simulink model "task1_simulation"  (R2025b)
settings: Solver=FixedStepAuto  StartTime=0.0  StopTime=40  RelTol=1e-3
undefined symbols (not defined in the file): d, DiscIntNeverNeededParam, is_real_robot, k_theta, k_x, k_y, q_goal_task1, q_goal_task2, q_init, r, Ts, X, Y
libraries: robotlib x6, sharedtransform x1
settings Model: Creator=dallaliber  LastModifiedBy=ilia
settings OptimizationCC: DefaultParameterBehavior=Inlined  EnhancedBackFolding=on  PassReuseOutputArgsAs=Individual arguments  ZeroExternalMemoryAtStartup=off  ZeroInternalMemoryAtStartup=off  MaxStackSize=64  OptimizeBlockOrder=speed  DifferentSizesBufferReuse=on  OptimizationCustomize=off  EfficientTunableParamExpr=on
settings DebuggingCC: ParameterTunabilityLossMsg=error
settings HardwareCC: ProdBitPerPointer=32.0  ProdBitPerSizeT=32.0  ProdBitPerPtrDiffT=32.0  ProdLargestAtomicFloat=None  ProdIntDivRoundTo=Undefined  ProdEndianess=Unspecified  ProdWordSize=32.0  ProdHWDeviceType=Generic->Unspecified (assume 32-bit Generic)
settings SFSimCC: MATLABDynamicMemAlloc=off
settings RTWCC: SystemTargetFile=ert.tlc  HardwareBoard=Robot Operating System (ROS)  TLCOptions="-aInlineSetEventsForThisBaseRateFcn=TLC_FALSE -aSuppressMultiTaskScheduler=TLC_FALSE  -aRateBasedStepFcn=0"  TemplateMakefile=ert_default_tmf  Toolchain=Catkin  TargetLang=C++  Description=Embedded Coder
settings CodeAppCC: ForceParamTrailComments=on  IgnoreCustomStorageClasses=off  OperatorAnnotations=on  SimulinkDataObjDesc=on  SFDataObjDesc=on  InsertBlockDesc=on
settings ERTTargetCC: DynamicArrayContainerType=coder::array

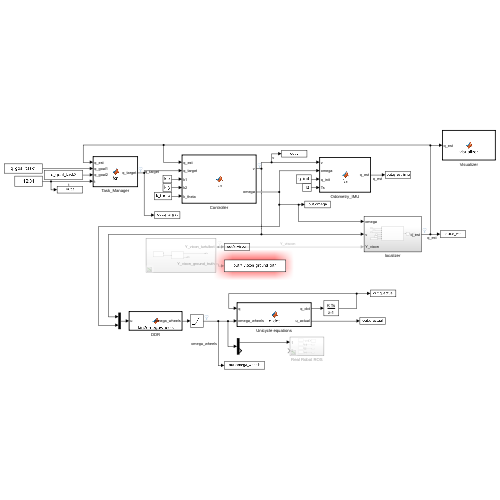
[thumbnail: Simulink's stored preview of the top-level diagram]
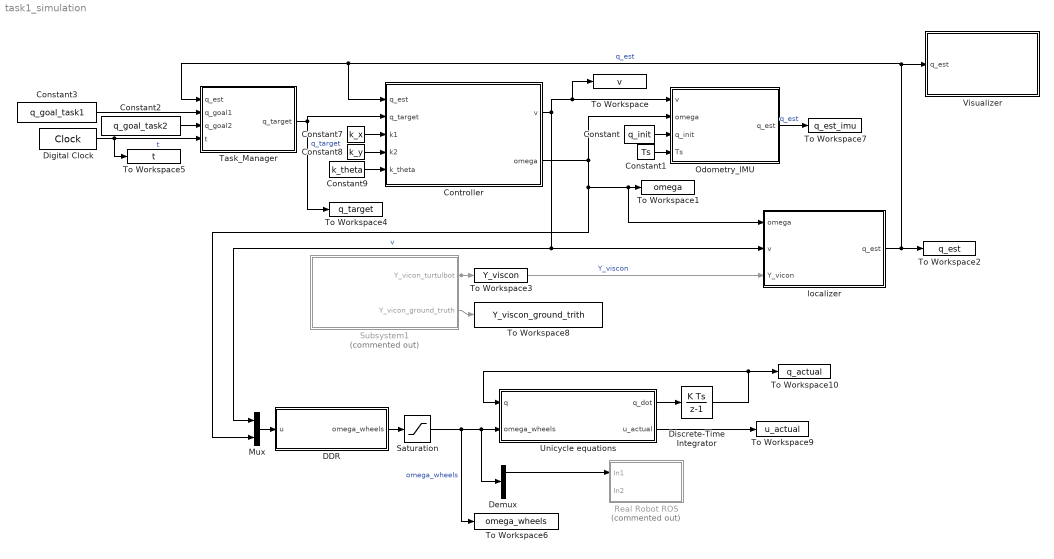
== system task1_simulation ==
  Constant : Constant  Value=q_init  SampleTime=Ts
  Constant1 : Constant  Value=Ts  SampleTime=Ts
  Constant2 : Constant  Value=q_goal_task2  SampleTime=Ts
  Constant3 : Constant  Value=q_goal_task1  SampleTime=Ts
  Constant7 : Constant  Value=k_x  SampleTime=Ts
  Constant8 : Constant  Value=k_y  SampleTime=Ts
  Constant9 : Constant  Value=k_theta  SampleTime=Ts
  Controller : MATLAB Function  TreatAsAtomicUnit=on
  DDR : MATLAB Function  TreatAsAtomicUnit=on
  Demux : Demux  Outputs=2
  Digital Clock : DigitalClock  SampleTime=Ts
  Discrete-Time Integrator : DiscreteIntegrator  InitialCondition=q_init  SampleTime=Ts  ICPrevOutput=DiscIntNeverNeededParam  ICPrevScaledInput=DiscIntNeverNeededParam
  Mux : Mux  Inputs=2
  Odometry_IMU : MATLAB Function  TreatAsAtomicUnit=on
  Real Robot ROS : Subsystem  Commented=on
  Saturation : Saturate  UpperLimit=10  LowerLimit=-10
  Subsystem1 : Subsystem  Commented=on
  Task_Manager : MATLAB Function  TreatAsAtomicUnit=on
  To Workspace : ToWorkspace  VariableName=v  SampleTime=Ts
  To Workspace1 : ToWorkspace  VariableName=omega  SampleTime=Ts
  To Workspace10 : ToWorkspace  VariableName=q_actual  SampleTime=Ts
  To Workspace2 : ToWorkspace  VariableName=q_est  SampleTime=Ts
  To Workspace3 : ToWorkspace  VariableName=Y_viscon  SampleTime=Ts
  To Workspace4 : ToWorkspace  VariableName=q_target  SampleTime=Ts
  To Workspace5 : ToWorkspace  VariableName=t  SampleTime=Ts
  To Workspace6 : ToWorkspace  VariableName=omega_wheels  SampleTime=Ts
  To Workspace7 : ToWorkspace  VariableName=q_est_imu  SampleTime=Ts
  To Workspace8 : ToWorkspace  VariableName=Y_viscon_ground_trith  SampleTime=Ts
  To Workspace9 : ToWorkspace  VariableName=u_actual  SampleTime=Ts
  Unicycle equations : MATLAB Function  TreatAsAtomicUnit=on
  Visualizer : MATLAB Function  TreatAsAtomicUnit=on
  localizer : Subsystem
  wires:
  Controller/1(v) -> Mux/1, localizer/2(v), Odometry_IMU/1(v), To Workspace/1  "v"
  Constant/1 -> Odometry_IMU/3(q_init)
  Constant1/1 -> Odometry_IMU/4(Ts)
  Constant2/1 -> Task_Manager/3(q_goal2)
  Constant3/1 -> Task_Manager/2(q_goal1)
  Odometry_IMU/1(q_est) -> To Workspace7/1  "q_est"
  Saturation/1 -> To Workspace6/1, Unicycle equations/2(omega_wheels), Demux/1  "omega_wheels"
  DDR/1(omega_wheels) -> Saturation/1
  Demux/1 -> Real Robot ROS/1(In1)
  Mux/1 -> DDR/1(u)
  Digital Clock/1 -> To Workspace5/1, Task_Manager/4(t)  "t"
  localizer/1(q_est) -> To Workspace2/1, Controller/1(q_est), Task_Manager/1(q_est), Visualizer/1(q_est)  "q_est"
  Subsystem1/1(Y_vicon_turtulbot) -> localizer/3(Y_vicon), To Workspace3/1  "Y_viscon"
  Task_Manager/1(q_target) -> To Workspace4/1, Controller/2(q_target)  "q_target"
  Constant7/1 -> Controller/3(k1)
  Constant8/1 -> Controller/4(k2)
  Subsystem1/2(Y_vicon_ground_truth) -> To Workspace8/1
  Constant9/1 -> Controller/5(k_theta)
  Controller/2(omega) -> localizer/1(omega), To Workspace1/1, Mux/2, Odometry_IMU/2(omega)
  Unicycle equations/1(q_dot) -> Discrete-Time Integrator/1
  Discrete-Time Integrator/1 -> To Workspace10/1, Unicycle equations/1(q)
  Unicycle equations/2(u_actual) -> To Workspace9/1

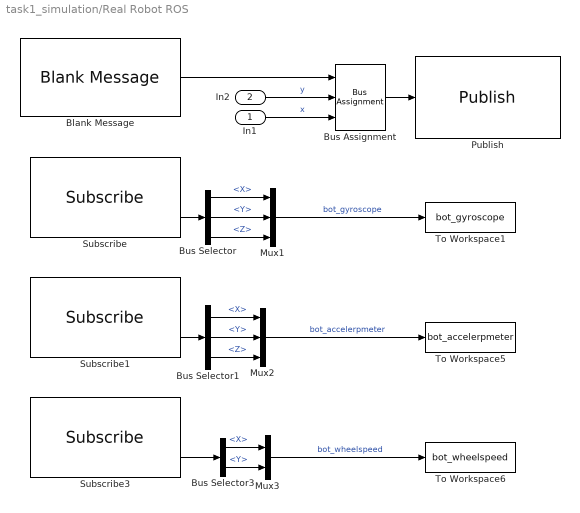
== system task1_simulation/Real Robot ROS ==
  In1 : Inport
  In2 : Inport  Port=2
  Blank Message : robotlib/Blank Message  messageClass=Message  entityType=geometry_msgs/Vector3  messageType=geometry_msgs/Vector3  SampleTime=0.04  legacyBusStruct=off
  Bus Assignment : BusAssignment  AssignedSignals=X,Y
  Bus Selector : BusSelector  OutputSignals=X,Y,Z
  Bus Selector1 : BusSelector  OutputSignals=X,Y,Z
  Bus Selector3 : BusSelector  OutputSignals=X,Y
  Mux1 : Mux  Inputs=3
  Mux2 : Mux  Inputs=3
  Mux3 : Mux  Inputs=2
  Publish : robotlib/Publish  topicSource=Select from ROS network  topic=/turtlebot_09/cmd_wheels  messageType=geometry_msgs/Vector3  legacyBusStruct=off  messageQueueLength=1
  Subscribe : robotlib/Subscribe  topicSource=Select from ROS network  topic=/turtlebot_09/gyroscope  messageType=geometry_msgs/Vector3  SampleTime=0.04  legacyBusStruct=off  messageQueueLength=1
  Subscribe1 : robotlib/Subscribe  topicSource=Select from ROS network  topic=/turtlebot_09/accelerometer  messageType=geometry_msgs/Vector3  SampleTime=0.04  legacyBusStruct=off  messageQueueLength=1
  Subscribe3 : robotlib/Subscribe  topicSource=Select from ROS network  topic=/turtlebot_09/wheelSpeeds  messageType=geometry_msgs/Vector3  SampleTime=0.04  legacyBusStruct=off  messageQueueLength=1
  To Workspace1 : ToWorkspace  VariableName=bot_gyroscope  SaveFormat=Timeseries  SampleTime=Ts
  To Workspace5 : ToWorkspace  VariableName=bot_accelerpmeter  SaveFormat=Timeseries  SampleTime=Ts
  To Workspace6 : ToWorkspace  VariableName=bot_wheelspeed  SaveFormat=Timeseries  SampleTime=Ts
  wires:
  Subscribe1/2 -> Bus Selector1/1
  Bus Selector1/1 -> Mux2/1  "<X>"
  Mux2/1 -> To Workspace5/1  "bot_accelerpmeter"
  Bus Assignment/1 -> Publish/1
  Subscribe/2 -> Bus Selector/1
  Bus Selector/2 -> Mux1/2  "<Y>"
  Bus Selector/1 -> Mux1/1  "<X>"
  Bus Selector3/1 -> Mux3/1  "<X>"
  Bus Selector3/2 -> Mux3/2  "<Y>"
  Bus Selector1/3 -> Mux2/3  "<Z>"
  Bus Selector1/2 -> Mux2/2  "<Y>"
  Mux3/1 -> To Workspace6/1  "bot_wheelspeed"
  Mux1/1 -> To Workspace1/1  "bot_gyroscope"
  Subscribe3/2 -> Bus Selector3/1
  Blank Message/1 -> Bus Assignment/1
  Bus Selector/3 -> Mux1/3  "<Z>"
  In1/1 -> Bus Assignment/3  "x"
  In2/1 -> Bus Assignment/2  "y"

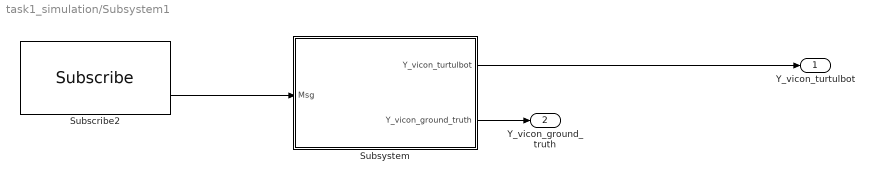
== system task1_simulation/Subsystem1 ==
  Subscribe2 : robotlib/Subscribe  topicSource=Select from ROS network  topic=/turtlebot_09/odom  messageType=nav_msgs/Odometry  SampleTime=Ts  legacyBusStruct=off  messageQueueLength=1
      settings: LibrarySourceBlock=roslib/ROS/Subscribe
  Subsystem : Subsystem
  Y_vicon_turtulbot : Outport
  Y_vicon_ground_truth : Outport  Port=2
  wires:
  Subscribe2/2 -> Subsystem/1(Msg)
  Subsystem/2(Y_vicon_ground_truth) -> Y_vicon_ground_truth/1
  Subsystem/1(Y_vicon_turtulbot) -> Y_vicon_turtulbot/1

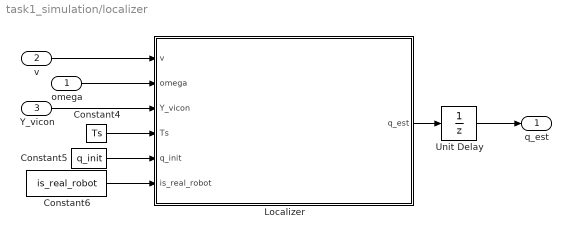
== system task1_simulation/localizer ==
  omega : Inport
  v : Inport  Port=2
  Y_vicon : Inport  Port=3
  Constant4 : Constant  Value=Ts
  Constant5 : Constant  Value=q_init
  Constant6 : Constant  Value=is_real_robot
  Localizer : MATLAB Function  TreatAsAtomicUnit=on
  Unit Delay : UnitDelay  InitialCondition=q_init  SampleTime=Ts  HasFrameUpgradeWarning=on
  q_est : Outport
  wires:
  Constant6/1 -> Localizer/6(is_real_robot)
  Y_vicon/1 -> Localizer/3(Y_vicon)
  Localizer/1(q_est) -> Unit Delay/1
  omega/1 -> Localizer/2(omega)
  Constant4/1 -> Localizer/4(Ts)
  Constant5/1 -> Localizer/5(q_init)
  Unit Delay/1 -> q_est/1
  v/1 -> Localizer/1(v)

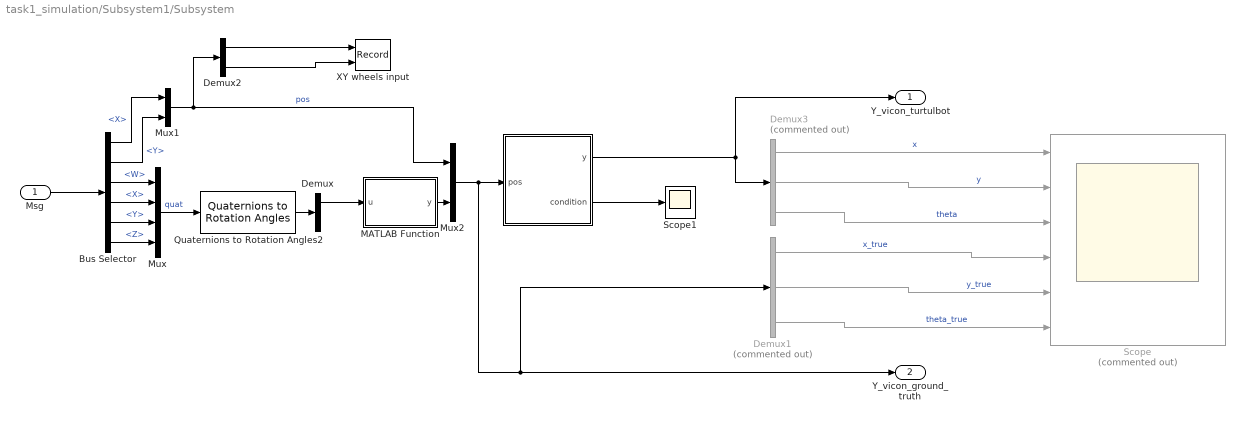
== system task1_simulation/Subsystem1/Subsystem ==
  Msg : Inport
  " " : MATLAB Function  TreatAsAtomicUnit=on
  Bus Selector : BusSelector  OutputSignals=Pose.Pose.Position.X,Pose.Pose.Position.Y,Pose.Pose.Orientation.W,Pose.Pose.Orientation.X,Pose.Pose.Orientation.Y,Pose.Pose.Orientation.Z
  Demux : Demux  Outputs=3
  Demux1 : Demux  Commented=on  Outputs=3
  Demux2 : Demux  Outputs=2
  Demux3 : Demux  Commented=on  Outputs=3
  MATLAB Function : MATLAB Function  TreatAsAtomicUnit=on
  Mux : Mux
  Mux1 : Mux  Inputs=2
  Mux2 : Mux  Inputs=2
  Quaternions to Rotation Angles2 : sharedtransform/Quaternions to Rotation Angles  rotationOrder=ZYX  aMode=aMode
  Scope : Scope  Commented=on  NumInputPorts=6
      settings: ActiveDisplayYMinimum=-0.22169  ActiveDisplayYMaximum=1.9952
  Scope1 : Scope
  XY wheels input : Record  NumPorts=2.0  FileSettingsInternal="{\"entries\":[{\"content\":{\"excelSettings\":{\"content\":{},\"type\":\"Streamout.ExcelSettings\"},\"parquetSettings\":{\"content\":{},\"type\":\"Streamout.ParquetSettings\"}},\"type\":\"Streamout.FileSettingStorage\",\"uuid\":\"\"}],\"packageUris\":[\"http:\\/\\/schema.mathworks.com\\/mf0\\/streamout_blocks\\/R2020a\"],\"version\":\"1.0\"}"  FrameSettings=[0, 0]  Layout=[1 1]  SignalsInternal="{\"entries\":[{\"content\":{\"signals\":[{\"content\":{\"blockPath\":[],\"dimensions\":[1],\"domain\":\"\",\"lineColor\":\"#7e2f8e\",\"lineWidth\":2,\"port\":1,\"signalID\":1,\"signalName\":\"Demux2:1\"},\"type\":\"RecordBlkView.Signal\",\"uuid\":\"\"},{\"content\":{\"blockPath\":[],\"dimensions\":[1],\"domain\":\"\",\"lineColor\":\"#77ac30\",\"lineWidth\":2,\"port\":2,\"signalID\":2,\"signalName\":\"Demux2:2\"},\"type\":\"RecordBlkView.Signal\",\"uuid\":\"\"}]},\"type\":\"RecordBlkView.InputSignals\",\"uuid\":\"\"}],\"packageUris\":[\"http:\\/\\/schema.mathworks.com\\/mf0\\/streamout_blocks\\/R2020a\"],\"version\":\"1.0\"}"  VisualizationBindings="{\"xyplotplugin\":{\"info\":[{\"series\":[],\"subplotID\":1}]}}"  CompatibilityTag=XY
  Y_vicon_turtulbot : Outport
  Y_vicon_ground_truth : Outport  Port=2
  wires:
  Msg/1 -> Bus Selector/1
  Mux2/1 -> Demux1/1, Y_vicon_ground_truth/1, " "/1(pos)
  Bus Selector/3 -> Mux/1  "<W>"
  Mux/1 -> Quaternions to Rotation Angles2/1  "quat"
  Bus Selector/2 -> Mux1/2  "<Y>"
  Demux3/1 -> Scope/1  "x"
  Bus Selector/6 -> Mux/4  "<Z>"
  Bus Selector/1 -> Mux1/1  "<X>"
  " "/1(y) -> Y_vicon_turtulbot/1, Demux3/1
  Demux1/2 -> Scope/5  "y_true"
  Bus Selector/4 -> Mux/2  "<X>"
  Bus Selector/5 -> Mux/3  "<Y>"
  Demux1/3 -> Scope/6  "theta_true"
  " "/2(condition) -> Scope1/1
  Demux3/3 -> Scope/3  "theta"
  Demux3/2 -> Scope/2  "y"
  Demux1/1 -> Scope/4  "x_true"
  MATLAB Function/1(y) -> Mux2/2
  Mux1/1 -> Demux2/1, Mux2/1  "pos"
  Quaternions to Rotation Angles2/1 -> Demux/1
  Demux/1 -> MATLAB Function/1(u)
  Demux2/1 -> XY wheels input/1
  Demux2/2 -> XY wheels input/2

== matlab function task1_simulation/Controller ==
  data: q_est input; v output; q_target input; k1 input; k2 input; k_theta input; omega output
function [v, omega] = fcn(q_est, q_target, k1, k2, k_theta)
    % Default outputs
    v = 0;
    omega = 0;
    
    % Internal safety limits
    v_limit = 0.22;       % linear velocity limit [m/s]
    omega_limit = 0.6;    % body angular velocity limit [rad/s]
                          % 10 rad/s is wheel-speed limit, not body omega
    
    % Position error
    dx = q_target(1) - q_est(1);
    dy = q_target(2) - q_est(2);
    
    rho = sqrt(dx^2 + dy^2);
    
    % ------------------------------------------------------------
    % Near target position: rotate in place to correct orientation
    % ------------------------------------------------------------
    if rho < 0.001
        e_theta = atan2(sin(q_target(3) - q_est(3)), ...
                        cos(q_target(3) - q_est(3)));
        
        v = 0;
        omega = k_theta * e_theta;
        
        % Saturate body angular velocity
        if abs(omega) > omega_limit
            omega = omega_limit * sign(omega);
        end
        
        % Stop only when orientation is also reached
        if abs(e_theta) < 0.05
            omega = 0;
        end
        
        return;
    end
    
    % Polar error variables
    theta_target = atan2(dy, dx);
    
    gamma = atan2(sin(theta_target - q_est(3)), ...
                  cos(theta_target - q_est(3)));
              
    delta = atan2(sin(gamma + q_est(3) - q_target(3)), ...
                  cos(gamma + q_est(3) - q_target(3)));
    
    % Astolfi posture regulation control law
    v = k1 * rho * cos(gamma);
    
    if abs(gamma) < 1e-4
        sinc_gamma = 1;
    else
        sinc_gamma = sin(gamma) / gamma;
    end
    
    omega = k2 * gamma + k1 * sinc_gamma * cos(gamma) * ...
            (gamma + k_theta * delta);
    
    % Saturation
    if abs(v) > v_limit
        v = v_limit * sign(v);
    end
    
    if abs(omega) > omega_limit
        omega = omega_limit * sign(omega);
    end
end

== matlab function task1_simulation/Odometry_IMU ==
  data: v input; q_est output; omega input; q_init input; Ts input
function q_est = fcn(v, omega, q_init, Ts)
    % Persistent variables hold their value between function calls
    persistent q_prev;
    
    if isempty(q_prev)
        q_prev = q_init;
    end
    
    % Dead-reckoning equations
    theta_new = q_prev(3) + omega * Ts;
    
    % Ensure angle is wrapped between -pi and pi
    theta_new = wrapToPi(theta_new);
    
    x_new = q_prev(1) + v * cos(theta_new) * Ts;
    y_new = q_prev(2) + v * sin(theta_new) * Ts;
    
    q_est = [x_new; y_new; theta_new];
    q_prev = q_est;
end

== matlab function task1_simulation/Visualizer ==
  data: q_est input
function visualizer(q_est)
    coder.extrinsic('draw_robot');
    draw_robot(q_est(1), q_est(2));
end

== matlab function task1_simulation/Subsystem1/Subsystem/  ==
  data: y output; pos input; condition output
function [y, condition] = check(pos)

x1 = -2.9; y1 = -1.5;
x2 = -1.6; y2 = -1.1;
x3 = -1.5; y3 = -0.7;
x4 = -1.4; y4 = -0.3;
x5 = -0.6; y5 =  0.1;
x6 =  0.2; y6 =  1.5;
x7 =  1.0;
x8 =  1.1;
x9 =  2.9;

P_loss = 0.9;


if ((pos(1) >= x5) && (pos(1) <= x6)) && ((pos(2) >= y1) && (pos(2) <= y5))
    % add noise
    y = pos + 0.02*randn(3,1);
    condition = 1;
elseif ((pos(1) >= x7) && (pos(1) <= x9)) && ((pos(2) >= y1) && (pos(2) <= y6))
    % measurement loss
    if rand > P_loss
        y = pos;
    else
        y = 0*pos;
    end
    condition = 2;
else
    y = pos;
    condition = 0;
end

== matlab function task1_simulation/localizer/Localizer ==
  data: v input; omega input; Y_vicon input; Ts input; q_est output; q_init input; is_real_robot input
function q_est = fcn(v, omega, Y_vicon, Ts, q_init, is_real_robot)
    % Extended Kalman Filter with Mode-Aware Initialization
    persistent q_hat P Q initialized
    
    % --- ۱. مقداردهی اولیه هوشمند ---
    if isempty(initialized)
        if is_real_robot == 1
            % در حالت واقعی: تا Vicon دیتا نداده، صبر کن
            if all(Y_vicon == 0)
                q_est = q_init; % یا خروجی فایلت را بده تا دیتا برسد
                return;
            else
                q_hat = Y_vicon; % اولین دیتای معتبر Vicon را قفل کن
                initialized = true;
            end
        else
            % در حالت شبیه‌سازی: بلافاصله با q_init استارت بزن
            q_hat = q_init;
            initialized = true;
        end
        P = eye(3) * 0.1; 
        Q = diag([1e-4, 1e-4, 5e-4]); % اعتماد به ادومتری
    end

    % --- ۲. پیش‌بینی (Prediction) ---
    theta = q_hat(3);
    % مدل کینماتیک غیرخطی یونیسایکل
    q_pred = q_hat + [v*cos(theta); v*sin(theta); omega] * Ts;
    q_pred(3) = wrapToPi(q_pred(3));

    % محاسبه ژاکوبیان (خطی‌سازی)
    F = [1, 0, -v*sin(theta)*Ts;
         0, 1,  v*cos(theta)*Ts;
         0, 0,  1];
    P = F * P * F' + Q;

    % --- ۳. اصلاح (Update) ---
    % تشخیص ناحیه قرمز (نویز سنسور)
    in_red = (q_pred(1) >= -0.6 && q_pred(1) <= 0.2);
    is_lost = all(Y_vicon == 0);

    if in_red
        R = diag([0.7, 0.7, 0.9]); % واریانس بالا برای ناحیه نویزی
    else
        R = diag([1e-5, 1e-5, 5e-5]); % واریانس پایین برای ناحیه امن
    end

    if is_lost
        % تسک ۳: سنسور قطع است، فقط ادومتری
        q_est = q_pred;
    else
        % فیلتر کالمن استاندارد
        H = eye(3);
        K = (P * H') / (H * P * H' + R);
        
        innovation = Y_vicon - q_pred;
        innovation(3) = wrapToPi(innovation(3)); % اصلاح زاویه در تفاضل
        
        q_est = q_pred + K * innovation;
        q_est(3) = wrapToPi(q_est(3));
        P = (eye(3) - K * H) * P;
    end
    
    q_hat = q_est;
end

== matlab function task1_simulation/Subsystem1/Subsystem/MATLAB Function ==
  data: u input; y output
function y = manual_unwrap(u)
    % این تابع به صورت دستی عملیات Unwrap را برای سیگنال‌های ورودی انجام می‌دهد.
    
    persistent prev_u cumulative_offset
    
    % مقداردهی اولیه در اولین گام اجرای شبیه‌سازی
    if isnan(u)
        u = 0;
    end
    if isempty(prev_u)
        prev_u = u;
        cumulative_offset = zeros(size(u));
    end
    
    % محاسبه اختلاف زاویه فعلی با قبلی
    diff = u - prev_u;
    
    % شناسایی پرش‌های بزرگتر از 180 درجه (pi رادیان)
    for i = 1:length(u)
        if diff(i) > pi
            cumulative_offset(i) = cumulative_offset(i) - 2*pi;
        elseif diff(i) < -pi
            cumulative_offset(i) = cumulative_offset(i) + 2*pi;
        end
    end
    
    % اعمال آفست تجمعی به ورودی فعلی
    y = u + cumulative_offset;
    
    % ذخیره مقدار فعلی برای استفاده در گام بعدی
    prev_u = u;

end

== matlab function task1_simulation/DDR ==
  data: u input; omega_wheels output; r parameter; d parameter
function omega_wheels = kin2omegawheels(u, r, d)
omega_l = u(1)/r-d/(2*r)*u(2);
omega_r = u(1)/r+d/(2*r)*u(2);
omega_wheels = [omega_l;omega_r];

== matlab function task1_simulation/Unicycle equations ==
  data: q input; omega_wheels input; q_dot output; r parameter; d parameter; u_actual output
function [q_dot, u_actual] = q_dot(q, omega_wheels, r, d)
u_actual = [r/2, r/2;-r/d, r/d]*omega_wheels;
theta = q(3);
q_dot = [[cos(theta), 0];[sin(theta), 0];[0,1]]*u_actual;

== matlab function task1_simulation/Task_Manager ==
  data: q_est input; q_target output; q_goal1 input; q_goal2 input; t input
function q_target = fcn(q_est, q_goal1, q_goal2, t)
    %#ok<INUSD>
    q_target = q_goal1;
end
